simulink model "DP_STD_MDL_DCAC_inv_2022b"  (R2022b)
settings: Solver=VariableStepAuto  StartTime=0.0  StopTime=6  RelTol=1e-3
libraries: spsSeriesRLCBranchLib x10, spsVoltageMeasurementLib x6, spsSecondOrderFilterLib x5, spsIdealSwitchLib x4, spsControlledVoltageSourceLib x2, peripheral_utilities x2, gmp_sil_core_pack x1, spsCurrentMeasurementLib x1, spspowerguiLib x1
settings Model: SimulationMode=accelerator  Creator=javnson  LastModifiedBy=javnson
settings DataIOCC: ReturnWorkspaceOutputs=off
settings OptimizationCC: ReuseModelBlockBuffer=on
settings RTWCC: GPUComputeCapability=5.0

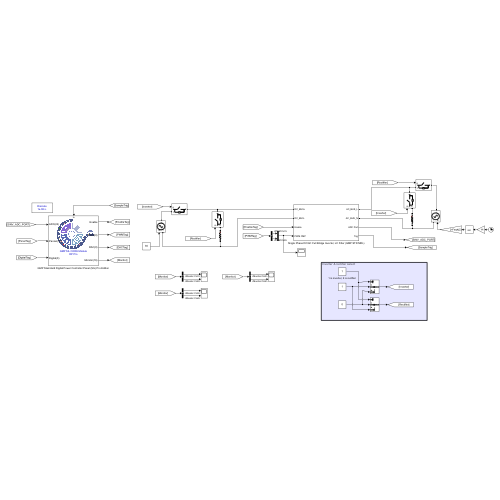
[thumbnail: Simulink's stored preview of the top-level diagram]
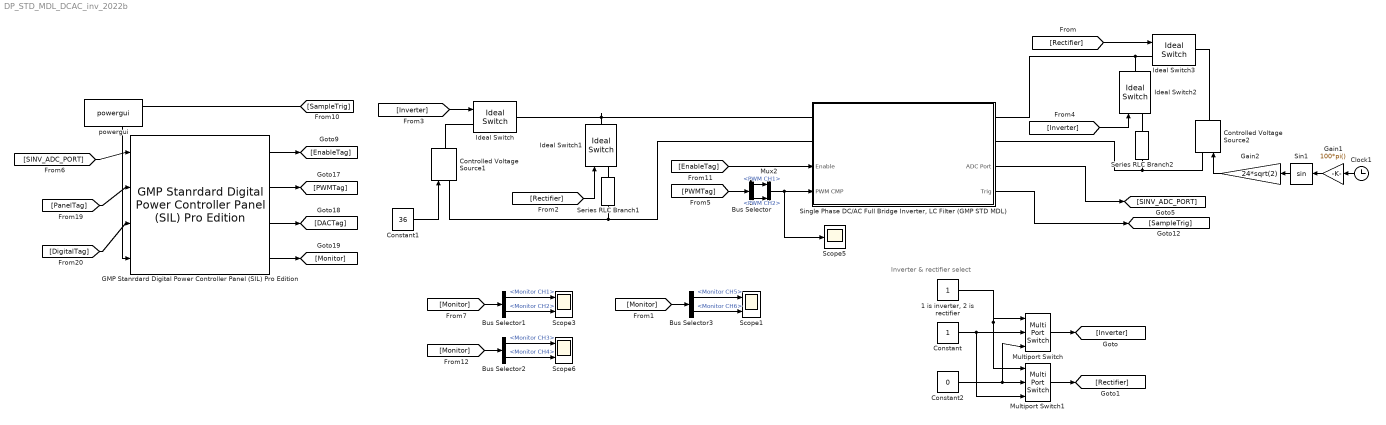
== system DP_STD_MDL_DCAC_inv_2022b ==
  note: Inverter & rectifier select
  "1 is inverter, 2 is rectifier" : Constant
  Bus Selector : BusSelector  OutputSignals=PWM CH1,PWM CH2
  Bus Selector1 : BusSelector  OutputSignals=Monitor CH1,Monitor CH2
  Bus Selector2 : BusSelector  OutputSignals=Monitor CH3,Monitor CH4
  Bus Selector3 : BusSelector  OutputSignals=Monitor CH5,Monitor CH6
  Clock1 : Clock
  Constant : Constant
  Constant1 : Constant  Value=36
  Constant2 : Constant  Value=0
  Controlled Voltage Source1 : spsControlledVoltageSourceLib/Controlled Voltage Source  Initialize=on  Source_Type=AC  Amplitude=0  Phase=0  Frequency=0  Measurements=None
  Controlled Voltage Source2 : spsControlledVoltageSourceLib/Controlled Voltage Source  Initialize=on  Source_Type=AC  Amplitude=0  Phase=0  Frequency=0  Measurements=None
  GMP Stanrdard Digital Power Controller Panel (SIL) Pro Edition : gmp_sil_core_pack/GMP Stanrdard Digital Power Controller Panel (SIL) Pro Edition
      settings: SourceProductName=GMP SIL Core Utilities
  Gain1 : Gain  Gain=100*pi()
  Gain2 : Gain  Gain=24*sqrt(2)
  Ideal Switch{,1..3} (4 alike) : spsIdealSwitchLib/Ideal Switch  Ron=0.001  Lon=0  IC=0  Rs=1e5  Cs=inf  Measurements=off
  Multiport Switch : MultiPortSwitch  Inputs=2  SaturateOnIntegerOverflow=off  InputSameDT=off
  Multiport Switch1 : MultiPortSwitch  Inputs=2  SaturateOnIntegerOverflow=off  InputSameDT=off
  Mux2 : Mux  Inputs=2
  Scope1 : Scope  NumInputPorts=2
  Scope3 : Scope  NumInputPorts=2
  Scope5 : Scope
  Scope6 : Scope  NumInputPorts=2
  Series RLC Branch1 : spsSeriesRLCBranchLib/Series RLC Branch  LConnTagsString=__new0  RConnTagsString=__new0  BranchType=R  Resistance=200  Inductance=1e-3  SetiL0=off  InitialCurrent=0  Capacitance=1e-6  Setx0=off  InitialVoltage=0  Measurements=None
  Series RLC Branch2 : spsSeriesRLCBranchLib/Series RLC Branch  LConnTagsString=__new0  RConnTagsString=__new0  BranchType=R  Resistance=18  Inductance=1e-3  SetiL0=off  InitialCurrent=0  Capacitance=1e-6  Setx0=off  InitialVoltage=0  Measurements=None
  Sin1 : Trigonometry
  "Single Phase DC/AC Full Bridge Inverter, LC Filter (GMP STD MDL)" : Subsystem  mask(Standard Single Phase DC/AC inverter / rectifier){R_mosfet_on=4.6e-3, Lon=0, Rd=0.01, Vf=0.5, Rs=1e5, Cs=inf, ACF_L=680e-6, ACF_L_ESR=0.05, ACF_C=22e-6, ACF_C_ESR=0.02, ACF_C_EPR=100e3, DC_CAP=680e-6*2, DC_CAP_ESR=0.09, DC_CAP_EPR=10e3, fswitch=20e3, CMP_MAX=5000, Deadband_Upper=100, Deadband_Lower=100, phase_shift=0, ADC_Resolution=12, DC_Voltage_Gain=3.3 / 203.3, DC_VOLTAGE_ADC_REFERENCE=2.5, DC_VOLTAGE_ADC_BIAS=0.9966, DC_VOLTAGE_ADC_CUT_FREQ=1.5e3, DC_BUS_CURRENT_SENSOR_R=0.005, DC_Current_Gain=20, DC_CURRENT_ADC_REFERENCE=2.5, DC_CURRENT_ADC_BIAS=0.9, DC_CURRENT_ADC_CUT_FREQ=1.5e3, AC_Voltage_Gain=3.3 / 203.3, AC_VOLTAGE_ADC_REFERENCE=2.5, AC_VOLTAGE_ADC_BIAS=0.9966, AC_VOLTAGE_ADC_CUT_FREQ=1.5e3, AC_Current_Gain=0.005 * 20, AC_CURRENT_ADC_REFERENCE=2.5, AC_CURRENT_ADC_BIAS=0.9, AC_CURRENT_ADC_INIT=0, CAP_CURRENT_SENSOR_R=0.005, CAP_Current_Gain=20, CAP_CURRENT_ADC_REFERENCE=2.5, CAP_CURRENT_ADC_BIAS=0.9, CAP_CURRENT_ADC_CUT_FREQ=1.5e3, GRID_CURRENT_SENSOR_R=0.005, Grid_Current_Gain=20, GRID_CURRENT_ADC_REFERENCE=2.5, GRID_CURRENT_ADC_BIAS=0.9, GRID_CURRENT_ADC_CUT_FREQ=1.5e3}
      mask prompts: ADC_Resolution "ADC_BIT:"; DC_Voltage_Gain "ADC_GAIN:"; DC_VOLTAGE_ADC_REFERENCE "ADC_REFERENCE:"; DC_VOLTAGE_ADC_BIAS "ADC_BIAS:"; DC_VOLTAGE_ADC_CUT_FREQ "cut_frequency:"; DC_Current_Gain "ADC_GAIN:"; DC_CURRENT_ADC_REFERENCE "ADC_REFERENCE:"; DC_CURRENT_ADC_BIAS "ADC_BIAS:"; DC_CURRENT_ADC_CUT_FREQ "ADC_FILTER:"; AC_Voltage_Gain "ADC_GAIN:"; AC_VOLTAGE_ADC_REFERENCE "ADC_REFERENCE:"; AC_VOLTAGE_ADC_BIAS "ADC_BIAS:"; AC_VOLTAGE_ADC_CUT_FREQ "cut_frequency:"; AC_Current_Gain "ADC_GAIN:"; AC_CURRENT_ADC_REFERENCE "ADC_REFERENCE:"; AC_CURRENT_ADC_BIAS "ADC_BIAS:"; AC_CURRENT_ADC_INIT "ADC_INIT:"; CAP_CURRENT_SENSOR_R "CAP_BUS_CURRENT_SENSOR_R:"; CAP_Current_Gain "ADC_GAIN:"; CAP_CURRENT_ADC_REFERENCE "ADC_REFERENCE:"; CAP_CURRENT_ADC_BIAS "ADC_BIAS:"; CAP_CURRENT_ADC_CUT_FREQ "ADC_FILTER:"; GRID_CURRENT_SENSOR_R "DC_BUS_CURRENT_SENSOR_R:"; Grid_Current_Gain "ADC_GAIN:"; GRID_CURRENT_ADC_REFERENCE "ADC_REFERENCE:"; GRID_CURRENT_ADC_BIAS "ADC_BIAS:"; GRID_CURRENT_ADC_CUT_FREQ "ADC_FILTER:"
      mask help: This module takes the inverter direction as the positive direction.
      settings: PortSchema="{\"entries\":[{\"content\":{\"sides\":[{\"content\":{\"connectorIds\":[\"LConn1\",\"LConn2\",\"In1\",\"In2\"]},\"type\":\"ConnectorPlacement.EquallySpacedRectSide\",\"uuid\":\"0e3e6e75-5e1a-455b-8a22-c69d0a4261ca\"},{\"content\":{\"connectorIds\":[\"RConn1\",\"RConn2\",\"Out1\",\"Out2\"],\"side\":\"RIGHT\"},\"type\":\"ConnectorPlacement.EquallySpacedRectSide\",\"uuid\":\"20326781-9238-4fea-80fd-ba96906d5d3f\"},{\"content\":{\"side\":\"TOP\"},\"type\":\"ConnectorPlacement.EquallySpacedRectSide\",\"uuid\":\"9e3289d3-0bee-4337-807b-c293a46cda9c\"}]},\"type\":\"ConnectorPlacement.EquallySpacedConnector\",\"uuid\":\"56bb35ad-d602-4874-b9bf-b95a81ef662c\"}],\"packageUris\":[\"http://schema.mathworks.com/mf0/Connector/R2020b\"],\"version\":\"1.0\"}"
      mask DialogControl ParameterGroupVar Prompt: 参数
      mask DialogControl Container4 Prompt: Component Parameters
      mask DialogControl Container7 Prompt: MOSFET
      mask DialogControl Control2 Prompt: Rds(on), unit Ohm
      mask DialogControl Control3 Prompt: Internal diode inducctance, unit H
      mask DialogControl Control4 Prompt: Internal diode resistance Rd, unit Ohm
      mask DialogControl Control5 Prompt: Internal diode forward voltage Vf, unit V
      mask DialogControl Control6 Prompt: Snubber resistance Rs, unit ohm
      mask DialogControl Control7 Prompt: Snubber Capacitance Cs, unit F
      mask DialogControl Container8 Prompt: LC Filter
      mask DialogControl Container20 Prompt: Filter Inductor
      mask DialogControl Control8 Prompt: AC Bus Filter Inductor (H)
      mask DialogControl Control42 Prompt: AC Bus Filter Inductor, ESR (Ohm)
      mask DialogControl Container21 Prompt: Filter Capcitor
      mask DialogControl Control43 Prompt: AC Bus Filter Capacitor (F)
      mask DialogControl Control44 Prompt: AC Bus Filter Capacitor, ESR (Ohm)
      mask DialogControl Control45 Prompt: AC Bus Filter Capacitor, EPR (Ohm)
      mask DialogControl Container22 Prompt: DC Bus Capacitor
      mask DialogControl Control46 Prompt: DC Bus Capacitor (F)
      mask DialogControl Control47 Prompt: DC Bus Capacitor, ESR (Ohm)
      mask DialogControl Control48 Prompt: DC Bus Capacitor, EPR (Ohm)
      mask DialogControl Container5 Prompt: PWM Parameers
      mask DialogControl Control9 Prompt: PWM Frequency (Hz):
      mask DialogControl Control10 Prompt: Full Scale PWM Compare value:
      mask DialogControl Control11 Prompt: (whole period is 2 * CMP_MAX ticks)
      mask DialogControl Control12 Prompt: Deadband Range Set (CMP Value):
      mask DialogControl Control13 Prompt: Single side deadband time: DEADBAND_CMP/2/CMP_MAX/fswitch
      mask DialogControl Control14 Prompt: Initial Phase Shift, unit rad
      mask DialogControl Container6 Prompt: ADC Parameters
      mask DialogControl Container14 Prompt: ADC Device
      mask DialogControl Control15 Prompt: ADC resolution:
      mask DialogControl Container15 Prompt: DC Side Voltage Sensor
      mask DialogControl Control16 Prompt: ADC Voltage Gain (Scale Factor):
      mask DialogControl Control17 Prompt: ADC reference Voltage(V)
      mask DialogControl Control18 Prompt: ADC Bias Voltage(V)
      mask DialogControl Control19 Prompt: Voltage Filter cut frequency (Hz):
      mask DialogControl Control20 Prompt: Generally, this value less than switch frequency / 10, greater than motor normal frequency * 3
      mask DialogControl Container16 Prompt: DC Side Current Sensor
      mask DialogControl Control26 Prompt: DC Bus Current Sensor Resistance
      mask DialogControl Control34 Prompt: ADC Current Gain (Scale Factor):
      mask DialogControl Control27 Prompt: ADC reference Voltage(V), ADC full scale current (when gain = 1)
      mask DialogControl Control28 Prompt: ADC Bias Current(A)
      mask DialogControl Control35 Prompt: Voltage Filter cut frequency (Hz):
      mask DialogControl Control36 Prompt: Generally, this value less than switch frequency / 10, greater than motor normal frequency * 3
      mask DialogControl Container17 Prompt: AC Side Voltage Sensor
      mask DialogControl Control16_copy Prompt: ADC Voltage Gain (Scale Factor):
      mask DialogControl Control17_copy Prompt: ADC reference Voltage(V)
      mask DialogControl Control18_copy Prompt: ADC Bias Voltage(V)
      mask DialogControl Control19_copy Prompt: Voltage Filter cut frequency (Hz):
      mask DialogControl Control20_copy Prompt: Generally, this value less than switch frequency / 10, greater than motor normal frequency * 3
      mask DialogControl Container18 Prompt: AC Side Current Sensor
      mask DialogControl Control26_copy Prompt: ADC Current Gain (Scale Factor):
      mask DialogControl Control27_copy Prompt: ADC reference Current(A), ADC full scale current (when gain = 1)
      mask DialogControl Control28_copy Prompt: ADC Bias Current(A)
      mask DialogControl Control29_copy Prompt: ADC initial Current Output(A)
      mask DialogControl Container19 Prompt: Capcitor Current Sensor
      mask DialogControl Control26_copy_copy Prompt: Filter Capacitor Current Sensor Resistance
      mask DialogControl Control34_copy Prompt: ADC Current Gain (Scale Factor):
      mask DialogControl Control27_copy_copy Prompt: ADC reference Voltage(V), ADC full scale current (when gain = 1)
      mask DialogControl Control28_copy_copy Prompt: ADC Bias Current(V)
      mask DialogControl Control35_copy Prompt: Voltage Filter cut frequency (Hz):
      mask DialogControl Control36_copy Prompt: Generally, this value less than switch frequency / 10, greater than motor normal frequency * 3
      mask DialogControl Container23 Prompt: Grid Current Sensor
      mask DialogControl Control26_copy_copy_copy Prompt: Grid Bus Current Sensor Resistance
      mask DialogControl Control34_copy_copy Prompt: ADC Current Gain (Scale Factor):
      mask DialogControl Control27_copy_copy_copy Prompt: ADC reference Voltage(V), ADC full scale current (when gain = 1)
      mask DialogControl Control28_copy_copy_copy Prompt: ADC Bias Current(V)
      mask DialogControl Control35_copy_copy Prompt: Voltage Filter cut frequency (Hz):
      mask DialogControl Control36_copy_copy Prompt: Generally, this value less than switch frequency / 10, greater than motor normal frequency * 3
  powergui : spspowerguiLib/powergui  Priority=1  SimulationMode=Discrete  SampleTime=1e-6  frequency=60  Iterations=50  frequencyindice=0  Pbase=100e6  ErrMax=1e-4  UnitsV=kV  UnitsW=MW  buscounter=0  FunctionMessages=off  echomessages=off  EnableUseOfTLC=off  CurrentSourceSwitches=off  DisableSnubberDevices=off  DisableRonSwitches=off  DisableVfSwitches=off  DisplayEquations=off  AutomaticDiscreteSolvers=off  SolverType=Tustin/Backward Euler (TBE)  Interpol=off  ExternalGateDelay=off  methode=off  Ts=100  x0status=blocks  SPID=on  SwTol=0  HookPort=off  NonlinearTolerance=1e-4  nMaxIteration=100  ContinueOnMaxIteration=off  RestoreLinks=warning  ResistiveCurrentMeasurement=off  Frange=[0:2:500]  Ylog=off  Xlog=on  ShowGrid=off  save=off  variable=ZData  structure=0  ZoomFFT=off  StartTime=0.0  cycles=1  DisplayStyle=1  fundamental=60  FreqAxis=off  MaxFrequency=1000  frequencyindicesteady=1  RmsSteady=1  display=off
  wires:
  Constant1/1 -> Controlled Voltage Source1/1
  [EnableTag] -> "Single Phase DC/AC Full Bridge Inverter, LC Filter (GMP STD MDL)"/1(Enable)
  "Single Phase DC/AC Full Bridge Inverter, LC Filter (GMP STD MDL)"/2(Trig) -> [SampleTrig]
  "Single Phase DC/AC Full Bridge Inverter, LC Filter (GMP STD MDL)"/1(ADC Port) -> [SINV_ADC_PORT]
  Gain1/1 -> Sin1/1
  Clock1/1 -> Gain1/1
  Sin1/1 -> Gain2/1
  Gain2/1 -> Controlled Voltage Source2/1
  [SampleTrig] -> GMP Stanrdard Digital Power Controller Panel (SIL) Pro Edition/4
  GMP Stanrdard Digital Power Controller Panel (SIL) Pro Edition/1 -> [EnableTag]
  GMP Stanrdard Digital Power Controller Panel (SIL) Pro Edition/2 -> [PWMTag]
  GMP Stanrdard Digital Power Controller Panel (SIL) Pro Edition/3 -> [DACTag]
  GMP Stanrdard Digital Power Controller Panel (SIL) Pro Edition/4 -> [Monitor]
  [SINV_ADC_PORT] -> GMP Stanrdard Digital Power Controller Panel (SIL) Pro Edition/1
  [PanelTag] -> GMP Stanrdard Digital Power Controller Panel (SIL) Pro Edition/2
  [DigitalTag] -> GMP Stanrdard Digital Power Controller Panel (SIL) Pro Edition/3
  [PWMTag] -> Bus Selector/1
  Bus Selector/1 -> Mux2/1  "<PWM CH1>"
  Bus Selector/2 -> Mux2/2  "<PWM CH2>"
  Mux2/1 -> Scope5/1, "Single Phase DC/AC Full Bridge Inverter, LC Filter (GMP STD MDL)"/2(PWM CMP)
  [Monitor] -> Bus Selector1/1
  Bus Selector1/1 -> Scope3/1  "<Monitor CH1>"
  Bus Selector1/2 -> Scope3/2  "<Monitor CH2>"
  [Monitor] -> Bus Selector2/1
  Bus Selector2/1 -> Scope6/1  "<Monitor CH3>"
  Bus Selector2/2 -> Scope6/2  "<Monitor CH4>"
  Bus Selector3/2 -> Scope1/2  "<Monitor CH6>"
  Bus Selector3/1 -> Scope1/1  "<Monitor CH5>"
  [Monitor] -> Bus Selector3/1
  [Rectifier] -> Ideal Switch3/1
  [Rectifier] -> Ideal Switch1/1
  [Inverter] -> Ideal Switch/1
  [Inverter] -> Ideal Switch2/1
  "1 is inverter, 2 is rectifier"/1 -> Multiport Switch/1, Multiport Switch1/1
  Constant/1 -> Multiport Switch/2, Multiport Switch1/3
  Constant2/1 -> Multiport Switch1/2, Multiport Switch/3
  Multiport Switch/1 -> [Inverter]
  Multiport Switch1/1 -> [Rectifier]
  connections:
  Ideal Switch/RConn1 -- Ideal Switch1/RConn1 -- "Single Phase DC/AC Full Bridge Inverter, LC Filter (GMP STD MDL)"/LConn1
  Controlled Voltage Source1/LConn1 -- Series RLC Branch1/RConn1 -- "Single Phase DC/AC Full Bridge Inverter, LC Filter (GMP STD MDL)"/LConn2
  Ideal Switch2/RConn1 -- "Single Phase DC/AC Full Bridge Inverter, LC Filter (GMP STD MDL)"/RConn1 -- Ideal Switch3/LConn1
  Controlled Voltage Source2/LConn1 -- Series RLC Branch2/RConn1 -- "Single Phase DC/AC Full Bridge Inverter, LC Filter (GMP STD MDL)"/RConn2
  Ideal Switch/LConn1 -- Controlled Voltage Source1/RConn1
  Series RLC Branch1/LConn1 -- Ideal Switch1/LConn1
  Ideal Switch2/LConn1 -- Series RLC Branch2/LConn1
  Ideal Switch3/RConn1 -- Controlled Voltage Source2/RConn1

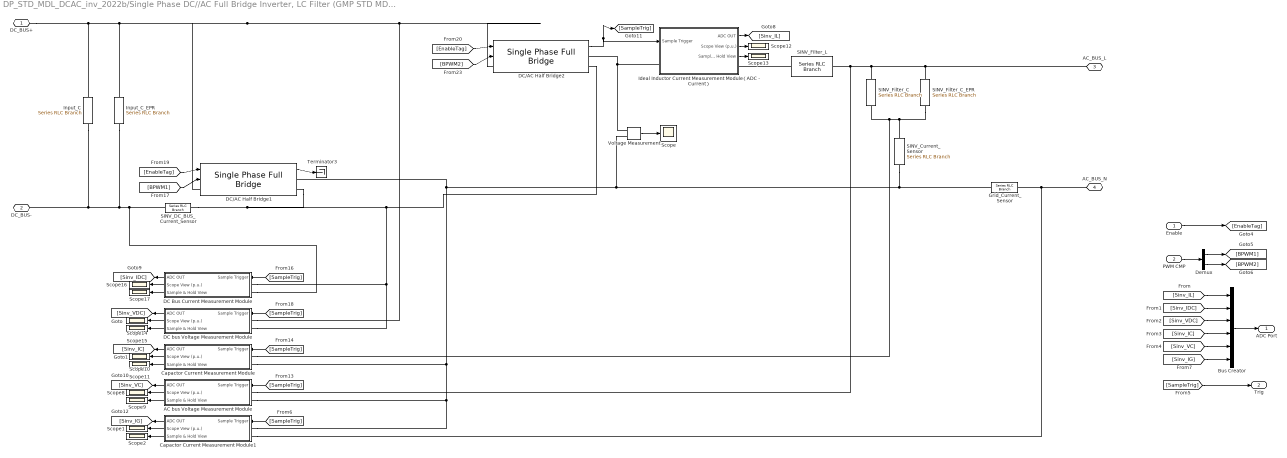
== system DP_STD_MDL_DCAC_inv_2022b/Single Phase DC//AC Full Bridge Inverter, LC Filter (GMP STD MDL) ==
  Enable : Inport
  PWM CMP : Inport  Port=2
  AC bus Voltage Measurement Module : Subsystem  AncestorBlock=peripheral_utilities/Ideal Voltage Measurement with filter Module(ADC - Voltage)  mask{ADC_GAIN=AC_Voltage_Gain, ADC_BIT=ADC_Resolution, ADC_REFERENCE=AC_VOLTAGE_ADC_REFERENCE, ADC_BIAS=AC_VOLTAGE_ADC_BIAS, ADC_INIT=0, cut_frequency=AC_VOLTAGE_ADC_CUT_FREQ}
      mask DialogControl DescGroupVar Prompt: Voltage Sample ADC Model
      mask DialogControl DescTextVar Prompt: This is a ideal Voltage Measurement Module.
      mask DialogControl Control2 Prompt: ADC(p.u.) = (real_voltage * ADC_GAIN + ADC_BIAS)/ADC_REFERENCE
      mask DialogControl Control11 Prompt: GMP CTL Simulink Utilities: virtual peripherals
      mask DialogControl ParameterGroupVar Prompt: Parameters:
      mask DialogControl Control4 Prompt: ADC Voltage Gain (Scale Factor):
      mask DialogControl Control5 Prompt: ADC resolution:
      mask DialogControl Control6 Prompt: ADC reference Voltage(V)
      mask DialogControl Control8 Prompt: ADC Bias Voltage(V)
      mask DialogControl Control7 Prompt: ADC Initial Voltage Output (V):
      mask DialogControl Control9 Prompt: Voltage Filter cut frequency (Hz):
      mask DialogControl Control10 Prompt: Generally, this value less than switch frequency / 10, greater than motor normal frequency * 3
  Bus Creator : BusCreator  Inputs=6
  Capactor Current Measurement Module : Subsystem  AncestorBlock=peripheral_utilities/Ideal Voltage Measurement with filter Module(ADC - Voltage)  mask{ADC_GAIN=CAP_Current_Gain, ADC_BIT=ADC_Resolution, ADC_REFERENCE=CAP_CURRENT_ADC_REFERENCE, ADC_BIAS=CAP_CURRENT_ADC_BIAS, ADC_INIT=0, cut_frequency=CAP_CURRENT_ADC_CUT_FREQ}
      mask DialogControl DescGroupVar Prompt: Voltage Sample ADC Model
      mask DialogControl DescTextVar Prompt: This is a ideal Voltage Measurement Module.
      mask DialogControl Control2 Prompt: ADC(p.u.) = (real_voltage * ADC_GAIN + ADC_BIAS)/ADC_REFERENCE
      mask DialogControl Control11 Prompt: GMP CTL Simulink Utilities: virtual peripherals
      mask DialogControl ParameterGroupVar Prompt: Parameters:
      mask DialogControl Control4 Prompt: ADC Voltage Gain (Scale Factor):
      mask DialogControl Control5 Prompt: ADC resolution:
      mask DialogControl Control6 Prompt: ADC reference Voltage(V)
      mask DialogControl Control8 Prompt: ADC Bias Voltage(V)
      mask DialogControl Control7 Prompt: ADC Initial Voltage Output (V):
      mask DialogControl Control9 Prompt: Voltage Filter cut frequency (Hz):
      mask DialogControl Control10 Prompt: Generally, this value less than switch frequency / 10, greater than motor normal frequency * 3
  Capactor Current Measurement Module1 : Subsystem  AncestorBlock=peripheral_utilities/Ideal Voltage Measurement with filter Module(ADC - Voltage)  mask{ADC_GAIN=Grid_Current_Gain, ADC_BIT=ADC_Resolution, ADC_REFERENCE=GRID_CURRENT_ADC_REFERENCE, ADC_BIAS=GRID_CURRENT_ADC_BIAS, ADC_INIT=0, cut_frequency=GRID_CURRENT_ADC_CUT_FREQ}
      mask DialogControl DescGroupVar Prompt: Voltage Sample ADC Model
      mask DialogControl DescTextVar Prompt: This is a ideal Voltage Measurement Module.
      mask DialogControl Control2 Prompt: ADC(p.u.) = (real_voltage * ADC_GAIN + ADC_BIAS)/ADC_REFERENCE
      mask DialogControl Control11 Prompt: GMP CTL Simulink Utilities: virtual peripherals
      mask DialogControl ParameterGroupVar Prompt: Parameters:
      mask DialogControl Control4 Prompt: ADC Voltage Gain (Scale Factor):
      mask DialogControl Control5 Prompt: ADC resolution:
      mask DialogControl Control6 Prompt: ADC reference Voltage(V)
      mask DialogControl Control8 Prompt: ADC Bias Voltage(V)
      mask DialogControl Control7 Prompt: ADC Initial Voltage Output (V):
      mask DialogControl Control9 Prompt: Voltage Filter cut frequency (Hz):
      mask DialogControl Control10 Prompt: Generally, this value less than switch frequency / 10, greater than motor normal frequency * 3
  DC Bus Current Measurement Module : Subsystem  AncestorBlock=peripheral_utilities/Ideal Voltage Measurement with filter Module(ADC - Voltage)  mask{ADC_GAIN=DC_Current_Gain, ADC_BIT=ADC_Resolution, ADC_REFERENCE=DC_CURRENT_ADC_REFERENCE, ADC_BIAS=DC_CURRENT_ADC_BIAS, ADC_INIT=0, cut_frequency=DC_CURRENT_ADC_CUT_FREQ}
      mask DialogControl DescGroupVar Prompt: Voltage Sample ADC Model
      mask DialogControl DescTextVar Prompt: This is a ideal Voltage Measurement Module.
      mask DialogControl Control2 Prompt: ADC(p.u.) = (real_voltage * ADC_GAIN + ADC_BIAS)/ADC_REFERENCE
      mask DialogControl Control11 Prompt: GMP CTL Simulink Utilities: virtual peripherals
      mask DialogControl ParameterGroupVar Prompt: Parameters:
      mask DialogControl Control4 Prompt: ADC Voltage Gain (Scale Factor):
      mask DialogControl Control5 Prompt: ADC resolution:
      mask DialogControl Control6 Prompt: ADC reference Voltage(V)
      mask DialogControl Control8 Prompt: ADC Bias Voltage(V)
      mask DialogControl Control7 Prompt: ADC Initial Voltage Output (V):
      mask DialogControl Control9 Prompt: Voltage Filter cut frequency (Hz):
      mask DialogControl Control10 Prompt: Generally, this value less than switch frequency / 10, greater than motor normal frequency * 3
  DC bus Voltage Measurement Module : Subsystem  AncestorBlock=peripheral_utilities/Ideal Voltage Measurement with filter Module(ADC - Voltage)  mask{ADC_GAIN=DC_Voltage_Gain, ADC_BIT=ADC_Resolution, ADC_REFERENCE=DC_VOLTAGE_ADC_REFERENCE, ADC_BIAS=DC_VOLTAGE_ADC_BIAS, ADC_INIT=0, cut_frequency=DC_VOLTAGE_ADC_CUT_FREQ}
      mask DialogControl DescGroupVar Prompt: Voltage Sample ADC Model
      mask DialogControl DescTextVar Prompt: This is a ideal Voltage Measurement Module.
      mask DialogControl Control2 Prompt: ADC(p.u.) = (real_voltage * ADC_GAIN + ADC_BIAS)/ADC_REFERENCE
      mask DialogControl Control11 Prompt: GMP CTL Simulink Utilities: virtual peripherals
      mask DialogControl ParameterGroupVar Prompt: Parameters:
      mask DialogControl Control4 Prompt: ADC Voltage Gain (Scale Factor):
      mask DialogControl Control5 Prompt: ADC resolution:
      mask DialogControl Control6 Prompt: ADC reference Voltage(V)
      mask DialogControl Control8 Prompt: ADC Bias Voltage(V)
      mask DialogControl Control7 Prompt: ADC Initial Voltage Output (V):
      mask DialogControl Control9 Prompt: Voltage Filter cut frequency (Hz):
      mask DialogControl Control10 Prompt: Generally, this value less than switch frequency / 10, greater than motor normal frequency * 3
  DC/AC Half Bridge1 : peripheral_utilities/Single Phase Full Bridge  fswitch=fswitch  CMP_MAX=CMP_MAX  Deadband_Upper=Deadband_Upper  Deadband_Lower=Deadband_Lower  Deadband_us=NaN  phase_shift=phase_shift  R_mosfet_on=R_mosfet_on  Lon=Lon  Rd=Rd  Vf=Vf  Rs=Rs  Cs=Cs
  DC/AC Half Bridge2 : peripheral_utilities/Single Phase Full Bridge  fswitch=fswitch  CMP_MAX=CMP_MAX  Deadband_Upper=Deadband_Upper  Deadband_Lower=Deadband_Lower  Deadband_us=NaN  phase_shift=phase_shift  R_mosfet_on=R_mosfet_on  Lon=Lon  Rd=Rd  Vf=Vf  Rs=Rs  Cs=Cs
  Demux : Demux  Outputs=2
  Grid_Current_Sensor : spsSeriesRLCBranchLib/Series RLC Branch  LConnTagsString=__new0  RConnTagsString=__new0  BranchType=R  Resistance=GRID_CURRENT_SENSOR_R  Inductance=1e-3  SetiL0=off  InitialCurrent=0  Capacitance=1e-6  Setx0=off  InitialVoltage=0  Measurements=None
  Ideal Inductor Current Measurement Module（ADC - Current） : Subsystem  AncestorBlock=peripheral_utilities/Ideal Current Measurement Module（ADC - Current）  mask{ADC_GAIN=AC_Current_Gain, ADC_BIT=ADC_Resolution, ADC_REFERENCE=AC_CURRENT_ADC_REFERENCE, ADC_BIAS=AC_CURRENT_ADC_BIAS, ADC_INIT=AC_CURRENT_ADC_INIT}
      mask DialogControl DescGroupVar Prompt: Current Sample ADC Model 1
      mask DialogControl DescTextVar Prompt: This is a ideal Current Measurement Module. This module enable a bias and a gain, and finally output a ADC result.
      mask DialogControl Control8 Prompt: ADC(p.u.) = (real_current * ADC_GAIN + ADC_BIAS)/ADC_REFERENCE
      mask DialogControl Control9 Prompt: GMP CTL Simulink Utilities: virtual peripherals
      mask DialogControl ParameterGroupVar Prompt: 参数
      mask DialogControl Control7 Prompt: ADC Current Gain (Scale Factor):
      mask DialogControl Control2 Prompt: ADC resolution:
      mask DialogControl Control4 Prompt: ADC reference Current(A), ADC full scale current (when gain = 1)
      mask DialogControl Control5 Prompt: ADC Bias Current(A)
      mask DialogControl Control6 Prompt: ADC initial Current Output(A)
  Input_C : spsSeriesRLCBranchLib/Series RLC Branch  LConnTagsString=__new0  RConnTagsString=__new0  BranchType=RC  Resistance=DC_CAP_ESR  Inductance=1e-3  SetiL0=off  InitialCurrent=0  Capacitance=DC_CAP  Setx0=off  InitialVoltage=0  Measurements=None
  Input_C_EPR : spsSeriesRLCBranchLib/Series RLC Branch  LConnTagsString=__new0  RConnTagsString=__new0  BranchType=R  Resistance=DC_CAP_EPR  Inductance=1e-3  SetiL0=off  InitialCurrent=0  Capacitance=1e-6  Setx0=off  InitialVoltage=0  Measurements=None
  SINV_Current_Sensor : spsSeriesRLCBranchLib/Series RLC Branch  LConnTagsString=__new0  RConnTagsString=__new0  BranchType=R  Resistance=CAP_CURRENT_SENSOR_R  Inductance=1e-3  SetiL0=off  InitialCurrent=0  Capacitance=1e-6  Setx0=off  InitialVoltage=0  Measurements=None
  SINV_DC_BUS_Current_Sensor : spsSeriesRLCBranchLib/Series RLC Branch  LConnTagsString=__new0  RConnTagsString=__new0  BranchType=R  Resistance=DC_BUS_CURRENT_SENSOR_R  Inductance=1e-3  SetiL0=off  InitialCurrent=0  Capacitance=1e-6  Setx0=off  InitialVoltage=0  Measurements=None
  SINV_Filter_C : spsSeriesRLCBranchLib/Series RLC Branch  LConnTagsString=__new0  RConnTagsString=__new0  BranchType=RC  Resistance=ACF_C_ESR  Inductance=1e-3  SetiL0=off  InitialCurrent=0  Capacitance=ACF_C  Setx0=off  InitialVoltage=0  Measurements=None
  SINV_Filter_C_EPR : spsSeriesRLCBranchLib/Series RLC Branch  LConnTagsString=__new0  RConnTagsString=__new0  BranchType=R  Resistance=ACF_C_EPR  Inductance=1e-3  SetiL0=off  InitialCurrent=0  Capacitance=1e-6  Setx0=off  InitialVoltage=0  Measurements=None
  SINV_Filter_L : spsSeriesRLCBranchLib/Series RLC Branch  LConnTagsString=__new0  RConnTagsString=__new0  BranchType=RL  Resistance=ACF_L_ESR  Inductance=ACF_L  SetiL0=off  InitialCurrent=0  Capacitance=1e-6  Setx0=off  InitialVoltage=0  Measurements=None
  Scope{,1..2,8..17} (13 alike) : Scope
  Terminator3 : Terminator
  Voltage Measurement : spsVoltageMeasurementLib/Voltage Measurement  PhasorSimulation=off  OutputType=Complex  PSBequivalent=0
  DC_BUS+ : PMIOPort  Side=Left
  DC_BUS- : PMIOPort  Port=2  Side=Left
  AC_BUS_L : PMIOPort  Port=3  Side=Right
  AC_BUS_N : PMIOPort  Port=4  Side=Right
  ADC Port : Outport
  Trig : Outport  Port=2
  wires:
  DC/AC Half Bridge2/1 -> Ideal Inductor Current Measurement Module（ADC - Current）/1(Sample Trigger), [SampleTrig]
  [BPWM2] -> DC/AC Half Bridge2/2
  AC bus Voltage Measurement Module/2(Scope View (p.u.)) -> Scope8/1
  AC bus Voltage Measurement Module/3(Sample & Hold View) -> Scope9/1
  [EnableTag] -> DC/AC Half Bridge2/1
  DC/AC Half Bridge1/1 -> Terminator3/1
  [SampleTrig] -> DC bus Voltage Measurement Module/1(Sample Trigger)
  Capactor Current Measurement Module/3(Sample & Hold View) -> Scope11/1
  [EnableTag] -> DC/AC Half Bridge1/1
  [SampleTrig] -> Capactor Current Measurement Module/1(Sample Trigger)
  [SampleTrig] -> AC bus Voltage Measurement Module/1(Sample Trigger)
  Capactor Current Measurement Module/2(Scope View (p.u.)) -> Scope10/1
  Capactor Current Measurement Module/1(ADC OUT) -> [Sinv_IC]
  AC bus Voltage Measurement Module/1(ADC OUT) -> [Sinv_VC]
  Ideal Inductor Current Measurement Module（ADC - Current）/3(Sample & Hold View) -> Scope13/1
  DC Bus Current Measurement Module/2(Scope View (p.u.)) -> Scope16/1
  Ideal Inductor Current Measurement Module（ADC - Current）/1(ADC OUT) -> [Sinv_IL]
  Ideal Inductor Current Measurement Module（ADC - Current）/2(Scope View (p.u.)) -> Scope12/1
  DC bus Voltage Measurement Module/2(Scope View (p.u.)) -> Scope14/1
  DC Bus Current Measurement Module/3(Sample & Hold View) -> Scope17/1
  [BPWM1] -> DC/AC Half Bridge1/2
  DC bus Voltage Measurement Module/3(Sample & Hold View) -> Scope15/1
  [SampleTrig] -> DC Bus Current Measurement Module/1(Sample Trigger)
  DC bus Voltage Measurement Module/1(ADC OUT) -> [Sinv_VDC]
  DC Bus Current Measurement Module/1(ADC OUT) -> [Sinv_IDC]
  Enable/1 -> [EnableTag]
  PWM CMP/1 -> Demux/1
  Demux/1 -> [BPWM1]
  Demux/2 -> [BPWM2]
  [Sinv_VDC] -> Bus Creator/3
  [Sinv_IDC] -> Bus Creator/2
  [Sinv_IL] -> Bus Creator/1
  [Sinv_IC] -> Bus Creator/4
  [Sinv_VC] -> Bus Creator/5
  Bus Creator/1 -> ADC Port/1
  [SampleTrig] -> Trig/1
  [SampleTrig] -> Capactor Current Measurement Module1/1(Sample Trigger)
  Capactor Current Measurement Module1/1(ADC OUT) -> [Sinv_IG]
  Capactor Current Measurement Module1/2(Scope View (p.u.)) -> Scope1/1
  Capactor Current Measurement Module1/3(Sample & Hold View) -> Scope2/1
  [Sinv_IG] -> Bus Creator/6
  Voltage Measurement/1 -> Scope/1
  connections:
  SINV_Filter_C/LConn1 -- AC bus Voltage Measurement Module/LConn1 -- SINV_Filter_L/RConn1 -- SINV_Filter_C_EPR/LConn1 -- AC_BUS_L/RConn1
  SINV_DC_BUS_Current_Sensor/RConn1 -- Input_C_EPR/RConn1 -- Input_C/RConn1 -- DC_BUS-/RConn1 -- DC Bus Current Measurement Module/LConn2
  DC Bus Current Measurement Module/LConn1 -- DC/AC Half Bridge2/RConn2 -- SINV_DC_BUS_Current_Sensor/LConn1 -- DC/AC Half Bridge1/RConn2 -- DC bus Voltage Measurement Module/LConn2
  SINV_Filter_C/RConn1 -- SINV_Filter_C_EPR/RConn1 -- SINV_Current_Sensor/LConn1 -- Capactor Current Measurement Module/LConn1
  Grid_Current_Sensor/LConn1 -- Capactor Current Measurement Module1/LConn2 -- AC_BUS_N/RConn1
  Input_C_EPR/LConn1 -- Input_C/LConn1 -- DC_BUS+/RConn1 -- DC/AC Half Bridge1/LConn1 -- DC/AC Half Bridge2/LConn1 -- DC bus Voltage Measurement Module/LConn1
  SINV_Filter_L/LConn1 -- Ideal Inductor Current Measurement Module（ADC - Current）/RConn1
  Ideal Inductor Current Measurement Module（ADC - Current）/LConn1 -- Voltage Measurement/LConn1 -- DC/AC Half Bridge2/RConn1
  Capactor Current Measurement Module/LConn2 -- Capactor Current Measurement Module1/LConn1 -- AC bus Voltage Measurement Module/LConn2 -- Voltage Measurement/LConn2 -- Grid_Current_Sensor/RConn1 -- SINV_Current_Sensor/RConn1 -- DC/AC Half Bridge1/RConn1

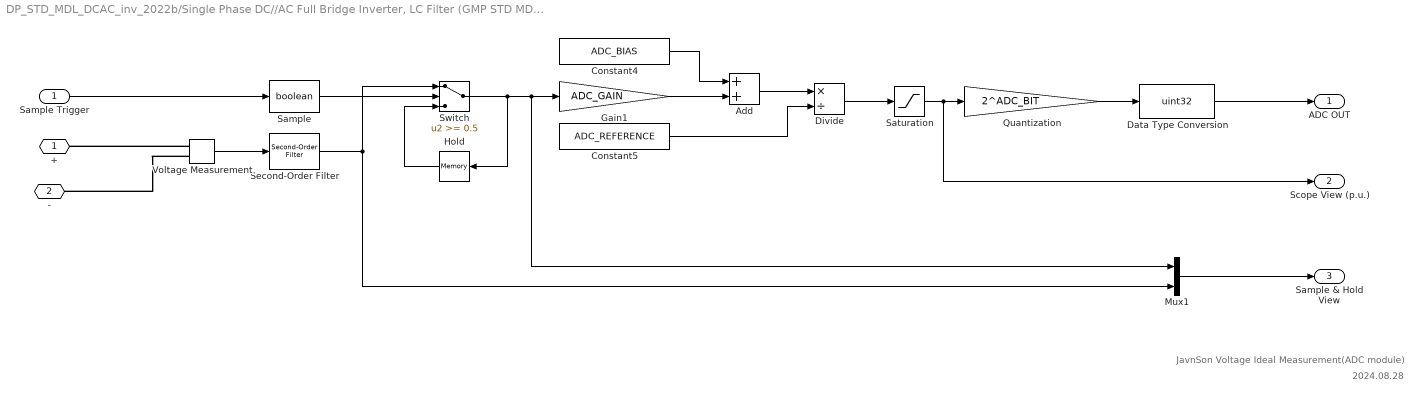
== system DP_STD_MDL_DCAC_inv_2022b/Single Phase DC//AC Full Bridge Inverter, LC Filter (GMP STD MDL)/AC bus Voltage Measurement Module ==
  note: 2024.08.28
  note: JavnSon Voltage Ideal Measurement(ADC module)
  Sample Trigger : Inport
  Add : Sum
  Constant4 : Constant  Value=ADC_BIAS
  Constant5 : Constant  Value=ADC_REFERENCE
  Data Type Conversion : DataTypeConversion  OutDataTypeStr=uint32  ConvertRealWorld=Stored Integer (SI)  SaturateOnIntegerOverflow=off  RndMeth=Floor
  Divide : Product  Inputs=*/
  Gain1 : Gain  Gain=ADC_GAIN
  Hold : Memory  InitialCondition=ADC_INIT  LinearizeAsDelay=on
  Mux1 : Mux  Inputs=2
  Quantization : Gain  Gain=2^ADC_BIT
  Sample : DataTypeConversion  OutDataTypeStr=boolean  SaturateOnIntegerOverflow=off  RndMeth=Floor
  Saturation : Saturate  UpperLimit=1  LowerLimit=0
  Second-Order Filter : spsSecondOrderFilterLib/Second-Order Filter  FilterType=Lowpass  Fo=cut_frequency  Zeta=0.707  Ts=0  Initialize=off  Vac_Init="[0,  0,  60]"  Vdc_Init=0  PlotResponse=off  FreqRange=[0, 500, 1]
  Switch : Switch  Threshold=0.5
  Voltage Measurement : spsVoltageMeasurementLib/Voltage Measurement  PhasorSimulation=off  OutputType=Complex  PSBequivalent=0
  + : PMIOPort  Side=Left
  - : PMIOPort  Port=2  Side=Left
  ADC OUT : Outport
  Scope View (p.u.) : Outport  Port=2
  Sample & Hold View : Outport  Port=3
  wires:
  Sample/1 -> Switch/2
  Add/1 -> Divide/1
  Constant5/1 -> Divide/2
  Quantization/1 -> Data Type Conversion/1
  Mux1/1 -> Sample & Hold View/1
  Data Type Conversion/1 -> ADC OUT/1
  Sample Trigger/1 -> Sample/1
  Gain1/1 -> Add/2
  Constant4/1 -> Add/1
  Saturation/1 -> Quantization/1, Scope View (p.u.)/1
  Voltage Measurement/1 -> Second-Order Filter/1
  Divide/1 -> Saturation/1
  Switch/1 -> Gain1/1, Mux1/1, Hold/1
  Hold/1 -> Switch/3
  Second-Order Filter/1 -> Switch/1, Mux1/2
  connections:
  Voltage Measurement/LConn2 -- -/RConn1
  Voltage Measurement/LConn1 -- +/RConn1

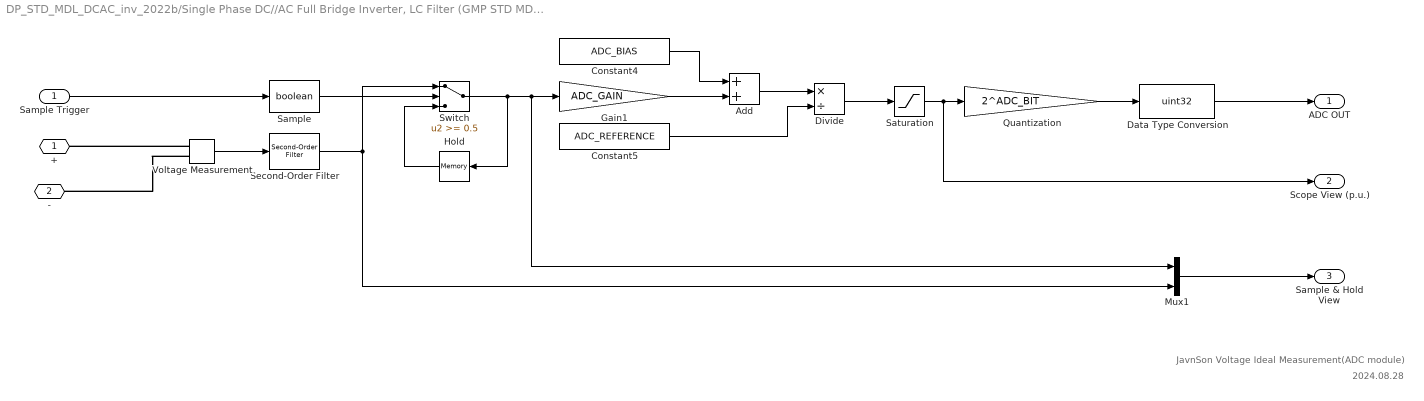
== system DP_STD_MDL_DCAC_inv_2022b/Single Phase DC//AC Full Bridge Inverter, LC Filter (GMP STD MDL)/Capactor Current Measurement Module ==
  note: JavnSon Voltage Ideal Measurement(ADC module)
  note: 2024.08.28
  Sample Trigger : Inport
  Add : Sum
  Constant4 : Constant  Value=ADC_BIAS
  Constant5 : Constant  Value=ADC_REFERENCE
  Data Type Conversion : DataTypeConversion  OutDataTypeStr=uint32  ConvertRealWorld=Stored Integer (SI)  SaturateOnIntegerOverflow=off  RndMeth=Floor
  Divide : Product  Inputs=*/
  Gain1 : Gain  Gain=ADC_GAIN
  Hold : Memory  InitialCondition=ADC_INIT  LinearizeAsDelay=on
  Mux1 : Mux  Inputs=2
  Quantization : Gain  Gain=2^ADC_BIT
  Sample : DataTypeConversion  OutDataTypeStr=boolean  SaturateOnIntegerOverflow=off  RndMeth=Floor
  Saturation : Saturate  UpperLimit=1  LowerLimit=0
  Second-Order Filter : spsSecondOrderFilterLib/Second-Order Filter  FilterType=Lowpass  Fo=cut_frequency  Zeta=0.707  Ts=0  Initialize=off  Vac_Init="[0,  0,  60]"  Vdc_Init=0  PlotResponse=off  FreqRange=[0, 500, 1]
  Switch : Switch  Threshold=0.5
  Voltage Measurement : spsVoltageMeasurementLib/Voltage Measurement  PhasorSimulation=off  OutputType=Complex  PSBequivalent=0
  + : PMIOPort  Side=Left
  - : PMIOPort  Port=2  Side=Left
  ADC OUT : Outport
  Scope View (p.u.) : Outport  Port=2
  Sample & Hold View : Outport  Port=3
  wires:
  Second-Order Filter/1 -> Mux1/2, Switch/1
  Hold/1 -> Switch/3
  Switch/1 -> Hold/1, Mux1/1, Gain1/1
  Divide/1 -> Saturation/1
  Voltage Measurement/1 -> Second-Order Filter/1
  Saturation/1 -> Scope View (p.u.)/1, Quantization/1
  Constant4/1 -> Add/1
  Gain1/1 -> Add/2
  Sample Trigger/1 -> Sample/1
  Data Type Conversion/1 -> ADC OUT/1
  Mux1/1 -> Sample & Hold View/1
  Quantization/1 -> Data Type Conversion/1
  Constant5/1 -> Divide/2
  Add/1 -> Divide/1
  Sample/1 -> Switch/2
  connections:
  Voltage Measurement/LConn1 -- +/RConn1
  Voltage Measurement/LConn2 -- -/RConn1

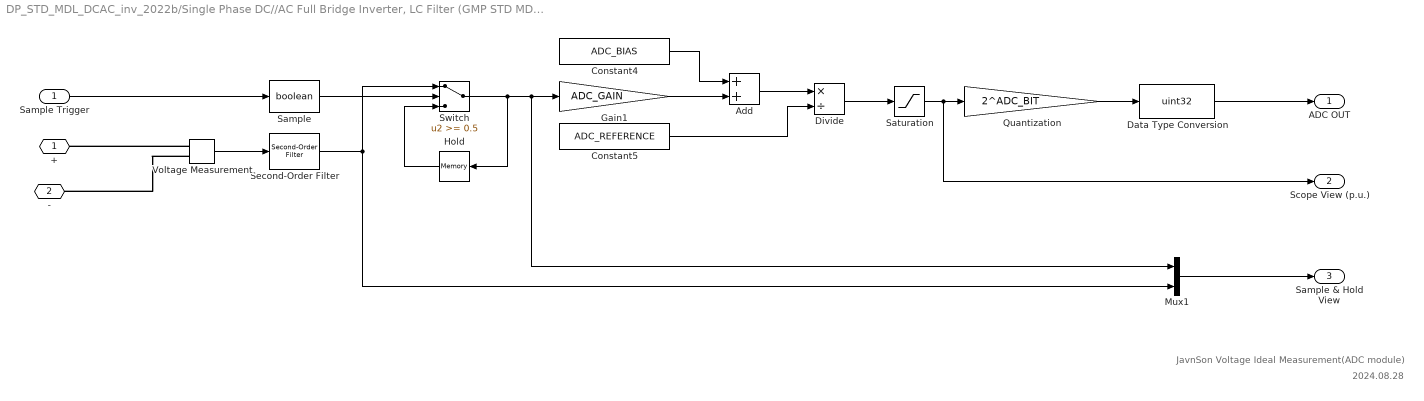
== system DP_STD_MDL_DCAC_inv_2022b/Single Phase DC//AC Full Bridge Inverter, LC Filter (GMP STD MDL)/Capactor Current Measurement Module1 ==
  note: 2024.08.28
  note: JavnSon Voltage Ideal Measurement(ADC module)
  Sample Trigger : Inport
  Add : Sum
  Constant4 : Constant  Value=ADC_BIAS
  Constant5 : Constant  Value=ADC_REFERENCE
  Data Type Conversion : DataTypeConversion  OutDataTypeStr=uint32  ConvertRealWorld=Stored Integer (SI)  SaturateOnIntegerOverflow=off  RndMeth=Floor
  Divide : Product  Inputs=*/
  Gain1 : Gain  Gain=ADC_GAIN
  Hold : Memory  InitialCondition=ADC_INIT  LinearizeAsDelay=on
  Mux1 : Mux  Inputs=2
  Quantization : Gain  Gain=2^ADC_BIT
  Sample : DataTypeConversion  OutDataTypeStr=boolean  SaturateOnIntegerOverflow=off  RndMeth=Floor
  Saturation : Saturate  UpperLimit=1  LowerLimit=0
  Second-Order Filter : spsSecondOrderFilterLib/Second-Order Filter  FilterType=Lowpass  Fo=cut_frequency  Zeta=0.707  Ts=0  Initialize=off  Vac_Init="[0,  0,  60]"  Vdc_Init=0  PlotResponse=off  FreqRange=[0, 500, 1]
  Switch : Switch  Threshold=0.5
  Voltage Measurement : spsVoltageMeasurementLib/Voltage Measurement  PhasorSimulation=off  OutputType=Complex  PSBequivalent=0
  + : PMIOPort  Side=Left
  - : PMIOPort  Port=2  Side=Left
  ADC OUT : Outport
  Scope View (p.u.) : Outport  Port=2
  Sample & Hold View : Outport  Port=3
  wires:
  Sample/1 -> Switch/2
  Add/1 -> Divide/1
  Constant5/1 -> Divide/2
  Quantization/1 -> Data Type Conversion/1
  Mux1/1 -> Sample & Hold View/1
  Data Type Conversion/1 -> ADC OUT/1
  Sample Trigger/1 -> Sample/1
  Gain1/1 -> Add/2
  Constant4/1 -> Add/1
  Saturation/1 -> Quantization/1, Scope View (p.u.)/1
  Voltage Measurement/1 -> Second-Order Filter/1
  Divide/1 -> Saturation/1
  Switch/1 -> Gain1/1, Mux1/1, Hold/1
  Hold/1 -> Switch/3
  Second-Order Filter/1 -> Switch/1, Mux1/2
  connections:
  Voltage Measurement/LConn2 -- -/RConn1
  Voltage Measurement/LConn1 -- +/RConn1

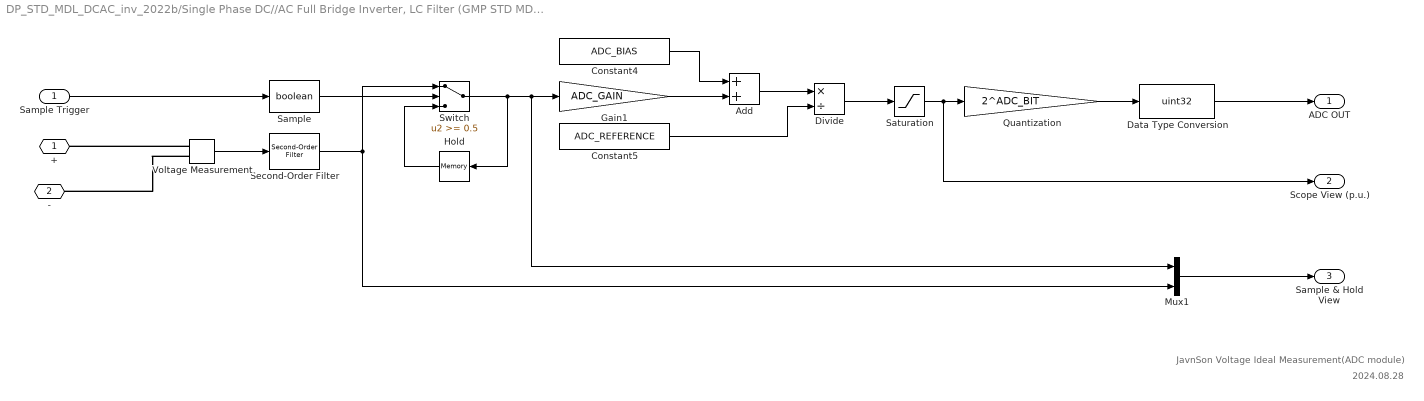
== system DP_STD_MDL_DCAC_inv_2022b/Single Phase DC//AC Full Bridge Inverter, LC Filter (GMP STD MDL)/DC Bus Current Measurement Module ==
  note: JavnSon Voltage Ideal Measurement(ADC module)
  note: 2024.08.28
  Sample Trigger : Inport
  Add : Sum
  Constant4 : Constant  Value=ADC_BIAS
  Constant5 : Constant  Value=ADC_REFERENCE
  Data Type Conversion : DataTypeConversion  OutDataTypeStr=uint32  ConvertRealWorld=Stored Integer (SI)  SaturateOnIntegerOverflow=off  RndMeth=Floor
  Divide : Product  Inputs=*/
  Gain1 : Gain  Gain=ADC_GAIN
  Hold : Memory  InitialCondition=ADC_INIT  LinearizeAsDelay=on
  Mux1 : Mux  Inputs=2
  Quantization : Gain  Gain=2^ADC_BIT
  Sample : DataTypeConversion  OutDataTypeStr=boolean  SaturateOnIntegerOverflow=off  RndMeth=Floor
  Saturation : Saturate  UpperLimit=1  LowerLimit=0
  Second-Order Filter : spsSecondOrderFilterLib/Second-Order Filter  FilterType=Lowpass  Fo=cut_frequency  Zeta=0.707  Ts=0  Initialize=off  Vac_Init="[0,  0,  60]"  Vdc_Init=0  PlotResponse=off  FreqRange=[0, 500, 1]
  Switch : Switch  Threshold=0.5
  Voltage Measurement : spsVoltageMeasurementLib/Voltage Measurement  PhasorSimulation=off  OutputType=Complex  PSBequivalent=0
  + : PMIOPort  Side=Left
  - : PMIOPort  Port=2  Side=Left
  ADC OUT : Outport
  Scope View (p.u.) : Outport  Port=2
  Sample & Hold View : Outport  Port=3
  wires:
  Second-Order Filter/1 -> Mux1/2, Switch/1
  Hold/1 -> Switch/3
  Switch/1 -> Hold/1, Mux1/1, Gain1/1
  Divide/1 -> Saturation/1
  Voltage Measurement/1 -> Second-Order Filter/1
  Saturation/1 -> Scope View (p.u.)/1, Quantization/1
  Constant4/1 -> Add/1
  Gain1/1 -> Add/2
  Sample Trigger/1 -> Sample/1
  Data Type Conversion/1 -> ADC OUT/1
  Mux1/1 -> Sample & Hold View/1
  Quantization/1 -> Data Type Conversion/1
  Constant5/1 -> Divide/2
  Add/1 -> Divide/1
  Sample/1 -> Switch/2
  connections:
  Voltage Measurement/LConn1 -- +/RConn1
  Voltage Measurement/LConn2 -- -/RConn1

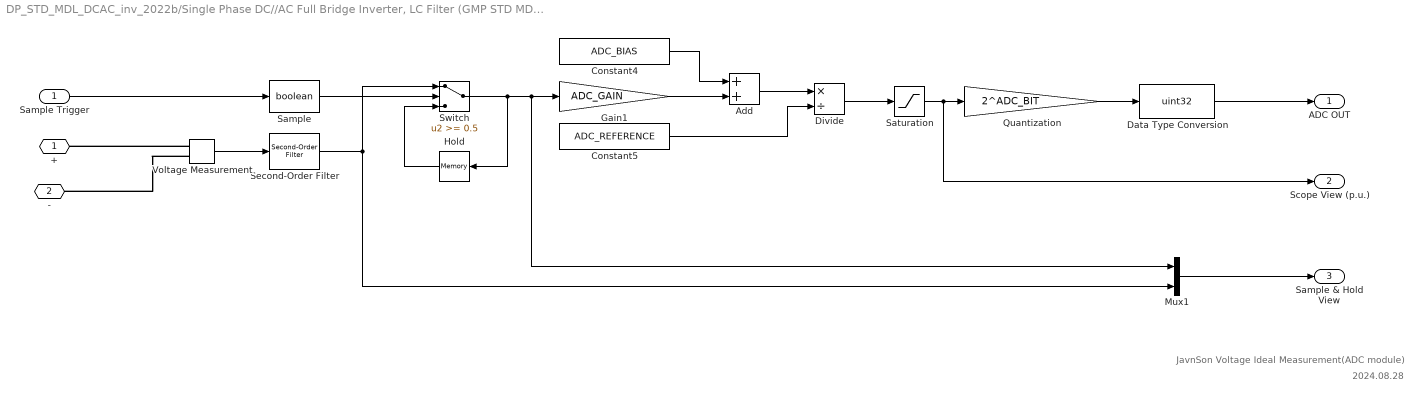
== system DP_STD_MDL_DCAC_inv_2022b/Single Phase DC//AC Full Bridge Inverter, LC Filter (GMP STD MDL)/DC bus Voltage Measurement Module ==
  note: 2024.08.28
  note: JavnSon Voltage Ideal Measurement(ADC module)
  Sample Trigger : Inport
  Add : Sum
  Constant4 : Constant  Value=ADC_BIAS
  Constant5 : Constant  Value=ADC_REFERENCE
  Data Type Conversion : DataTypeConversion  OutDataTypeStr=uint32  ConvertRealWorld=Stored Integer (SI)  SaturateOnIntegerOverflow=off  RndMeth=Floor
  Divide : Product  Inputs=*/
  Gain1 : Gain  Gain=ADC_GAIN
  Hold : Memory  InitialCondition=ADC_INIT  LinearizeAsDelay=on
  Mux1 : Mux  Inputs=2
  Quantization : Gain  Gain=2^ADC_BIT
  Sample : DataTypeConversion  OutDataTypeStr=boolean  SaturateOnIntegerOverflow=off  RndMeth=Floor
  Saturation : Saturate  UpperLimit=1  LowerLimit=0
  Second-Order Filter : spsSecondOrderFilterLib/Second-Order Filter  FilterType=Lowpass  Fo=cut_frequency  Zeta=0.707  Ts=0  Initialize=off  Vac_Init="[0,  0,  60]"  Vdc_Init=0  PlotResponse=off  FreqRange=[0, 500, 1]
  Switch : Switch  Threshold=0.5
  Voltage Measurement : spsVoltageMeasurementLib/Voltage Measurement  PhasorSimulation=off  OutputType=Complex  PSBequivalent=0
  + : PMIOPort  Side=Left
  - : PMIOPort  Port=2  Side=Left
  ADC OUT : Outport
  Scope View (p.u.) : Outport  Port=2
  Sample & Hold View : Outport  Port=3
  wires:
  Sample/1 -> Switch/2
  Add/1 -> Divide/1
  Constant5/1 -> Divide/2
  Quantization/1 -> Data Type Conversion/1
  Mux1/1 -> Sample & Hold View/1
  Data Type Conversion/1 -> ADC OUT/1
  Sample Trigger/1 -> Sample/1
  Gain1/1 -> Add/2
  Constant4/1 -> Add/1
  Saturation/1 -> Quantization/1, Scope View (p.u.)/1
  Voltage Measurement/1 -> Second-Order Filter/1
  Divide/1 -> Saturation/1
  Switch/1 -> Gain1/1, Mux1/1, Hold/1
  Hold/1 -> Switch/3
  Second-Order Filter/1 -> Switch/1, Mux1/2
  connections:
  Voltage Measurement/LConn2 -- -/RConn1
  Voltage Measurement/LConn1 -- +/RConn1

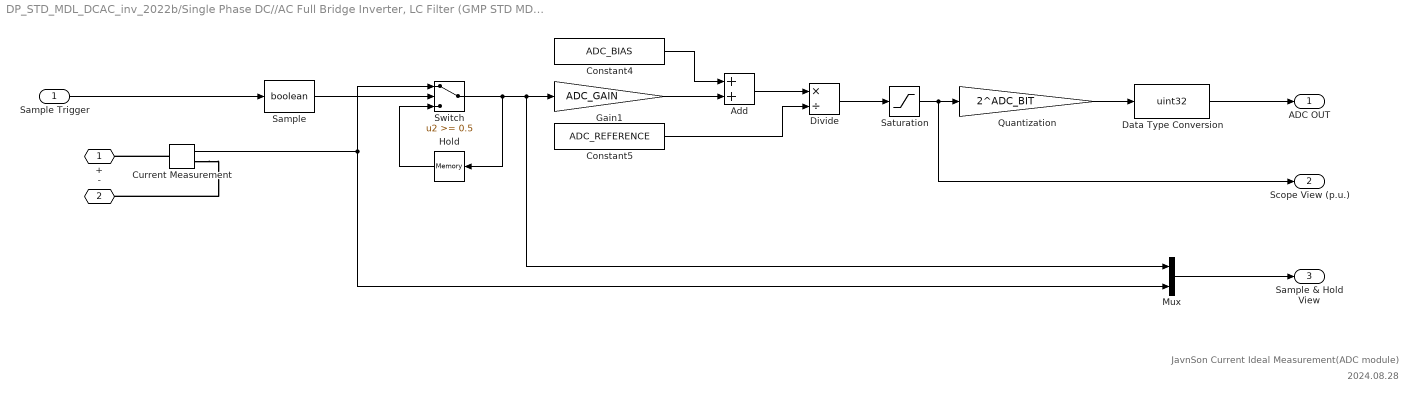
== system DP_STD_MDL_DCAC_inv_2022b/Single Phase DC//AC Full Bridge Inverter, LC Filter (GMP STD MDL)/Ideal Inductor Current Measurement Module（ADC - Current） ==
  note: 2024.08.28
  note: JavnSon Current Ideal Measurement(ADC module)
  Sample Trigger : Inport
  Add : Sum
  Constant4 : Constant  Value=ADC_BIAS
  Constant5 : Constant  Value=ADC_REFERENCE
  Current Measurement : spsCurrentMeasurementLib/Current Measurement  PhasorSimulation=off  OutputType=Complex  PSBequivalent=0
  Data Type Conversion : DataTypeConversion  OutDataTypeStr=uint32  ConvertRealWorld=Stored Integer (SI)  SaturateOnIntegerOverflow=off  RndMeth=Floor
  Divide : Product  Inputs=*/
  Gain1 : Gain  Gain=ADC_GAIN
  Hold : Memory  InitialCondition=ADC_INIT  LinearizeAsDelay=on
  Mux : Mux  Inputs=2
  Quantization : Gain  Gain=2^ADC_BIT
  Sample : DataTypeConversion  OutDataTypeStr=boolean  SaturateOnIntegerOverflow=off  RndMeth=Floor
  Saturation : Saturate  UpperLimit=1  LowerLimit=0
  Switch : Switch  Threshold=0.5
  + : PMIOPort  Side=Left
  - : PMIOPort  Port=2  Side=Right
  ADC OUT : Outport
  Scope View (p.u.) : Outport  Port=2
  Sample & Hold View : Outport  Port=3
  wires:
  Mux/1 -> Sample & Hold View/1
  Divide/1 -> Saturation/1
  Saturation/1 -> Quantization/1, Scope View (p.u.)/1
  Gain1/1 -> Add/2
  Switch/1 -> Gain1/1, Mux/1, Hold/1
  Constant4/1 -> Add/1
  Current Measurement/1 -> Switch/1, Mux/2
  Hold/1 -> Switch/3
  Data Type Conversion/1 -> ADC OUT/1
  Sample Trigger/1 -> Sample/1
  Add/1 -> Divide/1
  Sample/1 -> Switch/2
  Quantization/1 -> Data Type Conversion/1
  Constant5/1 -> Divide/2
  connections:
  Current Measurement/RConn1 -- -/RConn1
  Current Measurement/LConn1 -- +/RConn1
